simulink model "RunPositionController"  (R2023a)
settings: Solver=FixedStepAuto  StartTime=0.0  StopTime=10  FixedStep=T  RelTol=1e-3
values from neighbouring files (symbols this model uses):
  T = x(3)    [PT1T.m]    (also in SystemID_Setup.m = 0.0001; squarefit_motor.mat = 0.0001)
  Ts = 0.0001    [squarefit.m]
undefined symbols (not defined in the file or in its folder): National_Instruments, PCIe
libraries: sldrtlib x3, simulink_extras x1, slpidlib x1
settings Model: SimulationMode=external  ExtModeTrigDuration=100001  Creator=EAL  LastModifiedBy=EAL
settings SolverCC: AlgebraicLoopSolver=TrustRegion
settings DebuggingCC: UnconnectedInputMsg=warning  UnconnectedOutputMsg=warning  UnconnectedLineMsg=warning
settings HardwareCC: ProdBitPerLong=64  ProdHWDeviceType=Intel->x86-64 (Linux 64)
settings ModelReferenceCC: EnableRefExpFcnMdlSchedulingChecks=on
settings RTWCC: Description=Simulink Desktop Real-Time  SystemTargetFile=sldrt.tlc  TemplateMakefile=sldrt.tmf  RTWCompilerOptimization=on  DLArmComputeVersion=19.05
settings CodeAppCC: MaxIdLength=95
settings SimulinkDesktopRealTimeCC: TargetLibSuffix=_sldrt.a  TargetPreCompLibLocation=C:\Program Files\MATLAB\R2023a\toolbox\sldrt\lib\win64

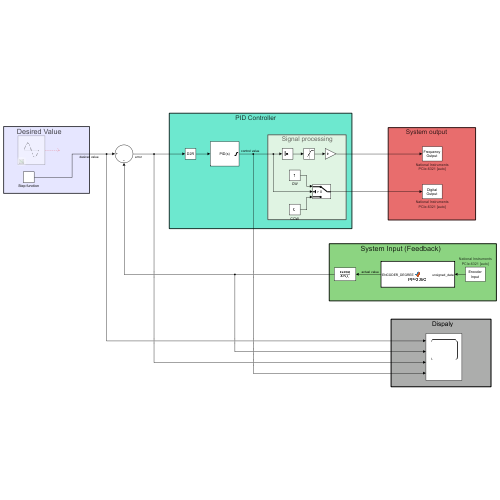
[thumbnail: Simulink's stored preview of the top-level diagram]
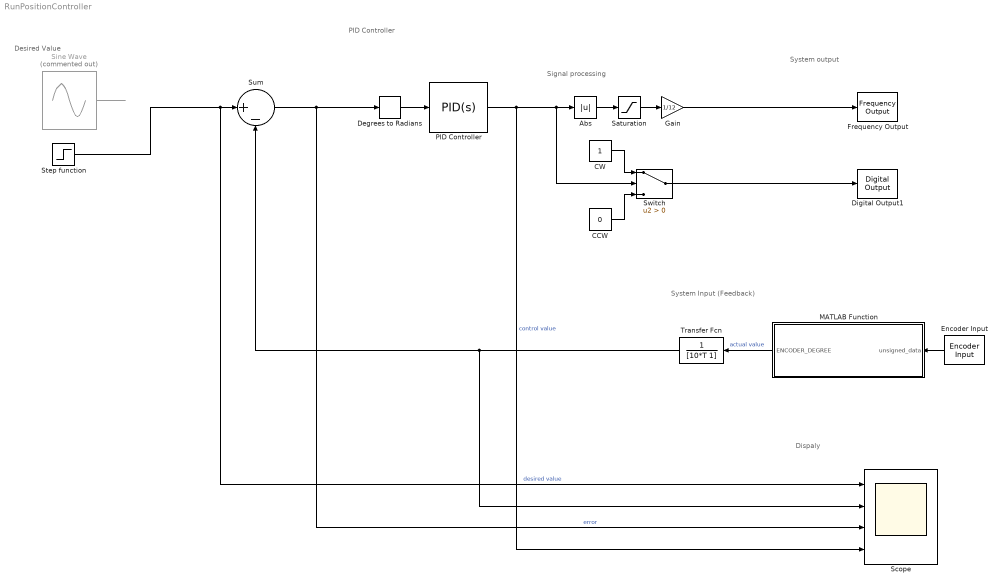
== system RunPositionController ==
  note: Desired Value
  note: System output
  note: Signal processing
  note: Dispaly
  note: System Input (Feedback)
  note: PID Controller
  Abs : Abs  SaturateOnIntegerOverflow=off
  CCW : Constant  Value=0
  CW : Constant
  Degrees to Radians : simulink_extras/Transformations/Degrees to Radians
  Digital Output1 : sldrtlib/Digital Output  SampleTime=Ts  MaxMissedTicks=1000000  ShowMissedTicks=off  YieldWhenWaiting=off  DrvName=National_Instruments/PCIe-6321  DrvAddress=4294967295  DrvOptions=[0 1 0 2 3 0 0]  Channels=1  BitMode=1  InitialValue=0  FinalValue=0
      settings: AttributesFormatString=National Instruments\nPCIe-6321 [auto]
  Encoder Input : sldrtlib/Encoder Input  SampleTime=Ts  MaxMissedTicks=100000  ShowMissedTicks=off  YieldWhenWaiting=off  DrvName=National_Instruments/PCIe-6321  DrvAddress=4294967295  DrvOptions=[0 1 0 2 3 0 0]  Channels=1  QuadMode=3  IndexPulse=1  InputFilter=Inf  DataType=1
      settings: AttributesFormatString=National Instruments\nPCIe-6321 [auto]
  Frequency Output : sldrtlib/Frequency Output  SampleTime=Ts  MaxMissedTicks=10000  ShowMissedTicks=off  YieldWhenWaiting=off  DrvName=National_Instruments/PCIe-6321  DrvAddress=4294967295  DrvOptions=[0 1 0 2 3 0 0]  Channels=2  FrequencySource=1  Frequency=15000  FrequencyFinalValue=[]  DutySource=2  Duty=0  DutyFinalValue=0
      settings: AttributesFormatString=National Instruments\nPCIe-6321 [auto]
  Gain : Gain  Gain=1/12
  MATLAB Function : MATLAB Function  TreatAsAtomicUnit=on
  PID Controller : slpidlib/PID Controller  Controller=PID  Form=Parallel  TimeDomain=Continuous-time  UseExternalTs=off  SampleTime=-1  IntegratorMethod=Forward Euler  FilterMethod=Forward Euler  ControllerParametersSource=internal  P=195  I=2.2197e+01  UseKiTs=off  D=4.2827  N=100  UseFilter=on  TunerSelectOption=Transfer Function Based (PID Tuner App)  InitialConditionSource=internal  InitialConditionForIntegrator=0  InitialConditionForFilter=0  DifferentiatorICPrevScaledInput=0  ExternalReset=none  TrackingMode=off  Kt=1  LimitOutput=on  SatLimitsSource=internal  UpperSaturationLimit=12  LowerSaturationLimit=-12  LinearizeAsGain=on  AntiWindupMode=clamping  Kb=1  LimitIntegrator=off  UpperIntegratorSaturationLimit=inf  LowerIntegratorSaturationLimit=-inf  POutMin=[]  POutMax=[]  IOutMin=[]  IOutMax=[]  DOutMin=[]  DOutMax=[]  NOutMin=[]  NOutMax=[]  SumOutMin=[]  SumOutMax=[]  SaturationOutMin=[]  SaturationOutMax=[]  PParamMin=[]  PParamMax=[]  IParamMin=[]  IParamMax=[]  DParamMin=[]  DParamMax=[]  NParamMin=[]  NParamMax=[]  KbParamMin=[]  KbParamMax=[]  KtParamMin=[]  KtParamMax=[]  KbOutMin=[]  KbOutMax=[]  KtOutMin=[]  KtOutMax=[]  IntegratorOutMin=[]  IntegratorOutMax=[]  FilterOutMin=[]  FilterOutMax=[]  SumI1OutMin=[]  SumI1OutMax=[]  SumI2OutMin=[]  SumI2OutMax=[]  SumI3OutMin=[]  SumI3OutMax=[]  SumI4OutMin=[]  SumI4OutMax=[]  SumDOutMin=[]  SumDOutMax=[]  DifferentiatorOutMin=[]  DifferentiatorOutMax=[]  FilterDiffOutCoefMin=[]  FilterDiffOutCoefMax=[]  ReciprocalOutMin=[]  ReciprocalOutMax=[]  SumDenOutMin=[]  SumDenOutMax=[]  SumNumOutMin=[]  SumNumOutMax=[]  DivideOutMin=[]  DivideOutMax=[]  UdiffTsProdOutMin=[]  UdiffTsProdOutMax=[]  NTsProdOutMin=[]  NTsProdOutMax=[]  UintegralTsProdOutMin=[]  UintegralTsProdOutMax=[]  UngainTsProdOutMin=[]  UngainTsProdOutMax=[]  ClampingZeroOutDataTypeStr=Inherit: Inherit via back propagation  ClampingZeroOutMin=[]  ClampingZeroOutMax=[]  FilterDenConstantOutDataTypeStr=Inherit: Inherit via back propagation  FilterDenConstantOutMin=[]  FilterDenConstantOutMax=[]  PCopyOutDataTypeStr=Inherit: Inherit via back propagation  PCopyOutMin=[]  PCopyOutMax=[]  NCopyOutDataTypeStr=Inherit: Inherit via back propagation  NCopyOutMin=[]  NCopyOutMax=[]  IntegratorContinuousStateAttributes=''  IntegratorStateMustResolveToSignalObject=off  IntegratorRTWStateStorageClass=Auto  FilterContinuousStateAttributes=''  FilterStateMustResolveToSignalObject=off  FilterRTWStateStorageClass=Auto  ParallelPVariant=InternalParameters  IdealPVariant=Disabled  IVariant=InternalParameters  DVariant=InternalParameters  IntegratorVariant=Continuous  SatVariant=Enabled  AWVariant=ContClampingParallel  PCopyVariant=Disabled  TRVariant=Disabled  FdbkBlocksVariant=Forward  IdealPFdbkVariant=Disabled  SatFdbkVariant=Disabled  DerivativeFilterVariant=ContFilter  NVariant=InternalParameters  NCopyVariant=Disabled  FilterICVariant=InternalICsFilter  IntegratorICVariant=InternalICs  ExternalResetVariant=Disabled  TRSumVariant=Passthrough  SumFdbkVariant=Disabled  SumVariant=Sum_PID  TsampFilterVariant=InternalTs  TsampNgainVariant=Passthrough  TsampIntegralVariant=Disabled_SignalSpec  ExternalSaturationOutDataTypeStr=Inherit: Same as second input
  Saturation : Saturate  UpperLimit=12  LowerLimit=0
  Scope : Scope  NumInputPorts=4
  Sine Wave : Sin  Commented=on  Amplitude=10  Frequency=5  SampleTime=0
  Step function : Step  Time=0  After=45  OutDataTypeStr=single
  Sum : Sum  Inputs=|+-
  Switch : Switch  Criteria=u2 > Threshold  SaturateOnIntegerOverflow=off  InputSameDT=off
  Transfer Fcn : TransferFcn  Denominator=[10*T 1]
  wires:
  Sine Wave/1 -> ?
  CCW/1 -> Switch/3
  PID Controller/1 -> Scope/4, Abs/1, Switch/2  "control value"
  Abs/1 -> Saturation/1
  Step function/1 -> Scope/1, Sum/1  "desired value"
  MATLAB Function/1(ENCODER_DEGREE) -> Transfer Fcn/1  "actual value"
  CW/1 -> Switch/1
  Degrees to Radians/1 -> PID Controller/1
  Encoder Input/1 -> MATLAB Function/1(unsigned_data)
  Saturation/1 -> Gain/1
  Sum/1 -> Scope/3, Degrees to Radians/1  "error"
  Gain/1 -> Frequency Output/1
  Switch/1 -> Digital Output1/1
  Transfer Fcn/1 -> Scope/2, Sum/2

== matlab function RunPositionController/MATLAB Function ==
  data: unsigned_data input; ENCODER_DEGREE output
function ENCODER_DEGREE = PPR2DEG(unsigned_data)
    ENCODER_PPR = 2000;
    COUNTER_N_BITS = 32;
    THRESHOLD = 2^(COUNTER_N_BITS - 1);
    if (unsigned_data > THRESHOLD)
        ENCODER_DEGREE = (unsigned_data - 2^COUNTER_N_BITS) * 360/ENCODER_PPR;
    else
        ENCODER_DEGREE = unsigned_data * 360/ENCODER_PPR;
    end

end
